simulink subsystem "Lqr"  (R2025b)
settings: Solver=VariableStepAuto
undefined symbols (not defined in the file): K_lqr_sim
settings Model: Creator=theha  LastModifiedBy=ahmed medhat

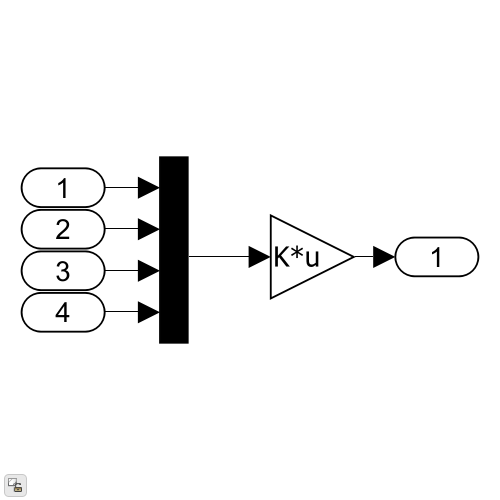
[thumbnail: Simulink's stored preview of the top-level diagram]
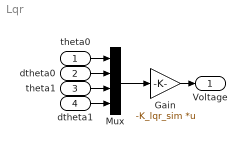
== system Lqr ==
  theta0 : Inport
  dtheta0 : Inport  Port=2
  theta1 : Inport  Port=3
  dtheta1 : Inport  Port=4
  Gain : Gain  Gain=-K_lqr_sim  Multiplication=Matrix(K*u)
  Mux : Mux
  Voltage : Outport
  wires:
  Mux/1 -> Gain/1
  dtheta0/1 -> Mux/2
  dtheta1/1 -> Mux/4
  Gain/1 -> Voltage/1
  theta0/1 -> Mux/1
  theta1/1 -> Mux/3
